simulink model "Planta"  (R2026b)
settings: Solver=VariableStepAuto
values from neighbouring files (symbols this model uses):
  b_m = 2e-6    (= 2e-06)    [Pendulo_Invertido.m]
  b_theta = 1e-3    (= 0.001)    [Pendulo_Invertido.m]
  b_x = 0.10    (= 0.1)    [Pendulo_Invertido.m]
  dtheta_init = 0    [Pendulo_Invertido.m]
  dx_init = 0    [Pendulo_Invertido.m]
  g = 9.80665    [Pendulo_Invertido.m]
  i_init = 0    [Pendulo_Invertido.m]
  Jp = m2*l*l + I    (= 0.024)    [Pendulo_Invertido.m]
  ke = kt    (= 0.0292)    [Pendulo_Invertido.m]
  kt = 0.0292    [Pendulo_Invertido.m]
  l = 0.30    (= 0.3)    [Pendulo_Invertido.m]
  La = 0.191e-3    (= 0.000191)    [Pendulo_Invertido.m]
  m2 = 0.20    (= 0.2)    [Pendulo_Invertido.m]
  Meq = M + Jm/(r*r)    (= 0.779)    [Pendulo_Invertido.m]
  r = 0.010    (= 0.01)    [Pendulo_Invertido.m]    (also in barrer_pid_theta.m = T(T.Kp==o.Kp(a)&T.Kd==o.Kd(b)&T.Ki==ki,:))
  Ra = 0.577    [Pendulo_Invertido.m]
  theta_init = pi - 20 * pi/180    (= 2.79252680319)    [Pendulo_Invertido.m]
  x_init = -0.35    [Pendulo_Invertido.m]
settings Model: Creator=fedeb  LastModifiedBy=fedeb

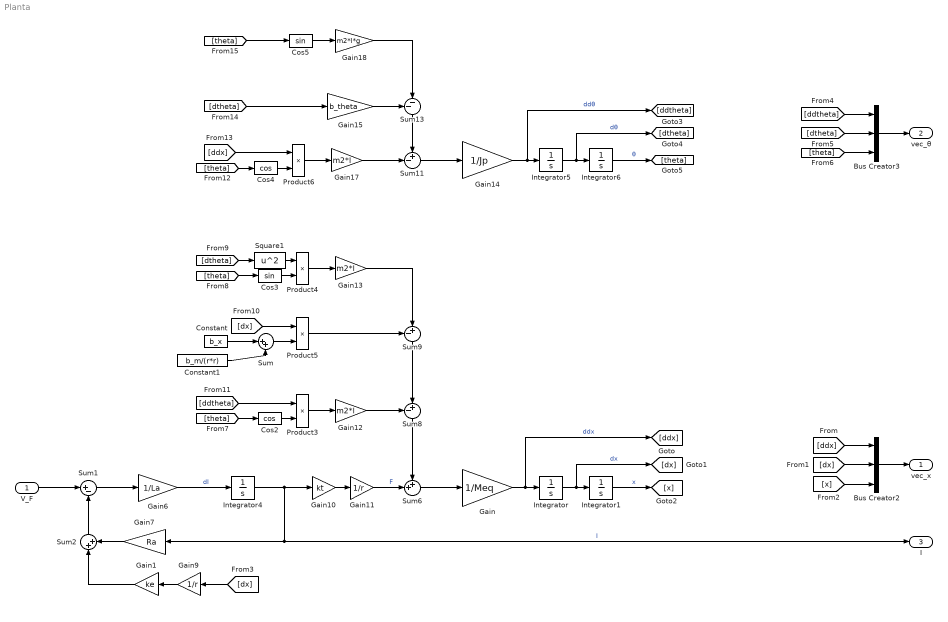
== system Planta ==
  V_F : Inport
  Bus Creator2 : BusCreator  Inputs=3
  Bus Creator3 : BusCreator  Inputs=3
  Constant : Constant  Value=b_x
  Constant1 : Constant  Value=b_m/(r*r)
  Cos2 : Trigonometry  Operator=cos
  Cos3 : Trigonometry
  Cos4 : Trigonometry  Operator=cos
  Cos5 : Trigonometry
  Gain : Gain  Gain=1/Meq
  Gain1 : Gain  Gain=ke
  Gain10 : Gain  Gain=kt
  Gain11 : Gain  Gain=1/r
  Gain12 : Gain  Gain=m2*l
  Gain13 : Gain  Gain=m2*l
  Gain14 : Gain  Gain=1/Jp
  Gain15 : Gain  Gain=b_theta
  Gain17 : Gain  Gain=m2*l
  Gain18 : Gain  Gain=m2*l*g
  Gain6 : Gain  Gain=1/La
  Gain7 : Gain  Gain=Ra
  Gain9 : Gain  Gain=1/r
  Integrator : Integrator  InitialCondition=dx_init
  Integrator1 : Integrator  InitialCondition=x_init
  Integrator4 : Integrator  InitialCondition=i_init
  Integrator5 : Integrator  InitialCondition=dtheta_init
  Integrator6 : Integrator  InitialCondition=theta_init
  Product{3..6} (4 alike) : Product
  Square1 : Math  Operator=square
  Sum : Sum  Inputs=|++
  Sum1 : Sum  Inputs=|+-
  Sum11 : Sum  Inputs=+-|
  Sum13 : Sum  Inputs=--|
  Sum2 : Sum  Inputs=|++
  Sum6 : Sum  Inputs=++|
  Sum8 : Sum  Inputs=-+|
  Sum9 : Sum  Inputs=-+|
  vec_x : Outport
  vec_θ : Outport  Port=2
  Ⅰ : Outport  Port=3
  wires:
  Integrator4/1 -> Gain10/1, Ⅰ/1, Gain7/1  "Ⅰ"
  V_F/1 -> Sum1/1
  Gain6/1 -> Integrator4/1  "dⅠ"
  Sum1/1 -> Gain6/1
  Gain7/1 -> Sum2/2
  Sum2/1 -> Sum1/2
  Gain1/1 -> Sum2/1
  Sum6/1 -> Gain/1
  Integrator/1 -> [dx], Integrator1/1  "dx"
  Integrator1/1 -> [x]  "x"
  Gain/1 -> [ddx], Integrator/1  "ddx"
  Gain10/1 -> Gain11/1
  Gain11/1 -> Sum6/2  "F"
  Bus Creator2/1 -> vec_x/1
  [ddx] -> Bus Creator2/1
  [dx] -> Bus Creator2/2
  [x] -> Bus Creator2/3
  Gain9/1 -> Gain1/1
  [dx] -> Gain9/1
  Sum8/1 -> Sum6/1
  Sum9/1 -> Sum8/2
  Gain12/1 -> Sum8/1
  Product3/1 -> Gain12/1
  Cos2/1 -> Product3/2
  Cos3/1 -> Product4/2
  Product4/1 -> Gain13/1
  Gain13/1 -> Sum9/2
  Square1/1 -> Product4/1
  Sum/1 -> Product5/2
  Product5/1 -> Sum9/1
  Constant/1 -> Sum/1
  Constant1/1 -> Sum/2
  Gain17/1 -> Sum11/2
  [dtheta] -> Bus Creator3/2
  Integrator6/1 -> [theta]  "θ"
  Gain18/1 -> Sum13/2
  Gain14/1 -> [ddtheta], Integrator5/1  "ddθ"
  Integrator5/1 -> [dtheta], Integrator6/1  "dθ"
  Cos4/1 -> Product6/2
  [theta] -> Bus Creator3/3
  Product6/1 -> Gain17/1
  Sum13/1 -> Sum11/1
  Sum11/1 -> Gain14/1
  [ddtheta] -> Bus Creator3/1
  Bus Creator3/1 -> vec_θ/1
  [theta] -> Cos2/1
  [theta] -> Cos3/1
  [dtheta] -> Square1/1
  [dx] -> Product5/1
  [ddtheta] -> Product3/1
  [theta] -> Cos4/1
  [ddx] -> Product6/1
  Gain15/1 -> Sum13/1
  [dtheta] -> Gain15/1
  Cos5/1 -> Gain18/1
  [theta] -> Cos5/1
